simulink subsystem "Wind_Forces"  (R2026a)
settings: Solver=VariableStepAuto
undefined symbols (not defined in the file): IN, pressureLevels, uwndTable, vwndTable
settings Model: Creator=asing  LastModifiedBy=asing

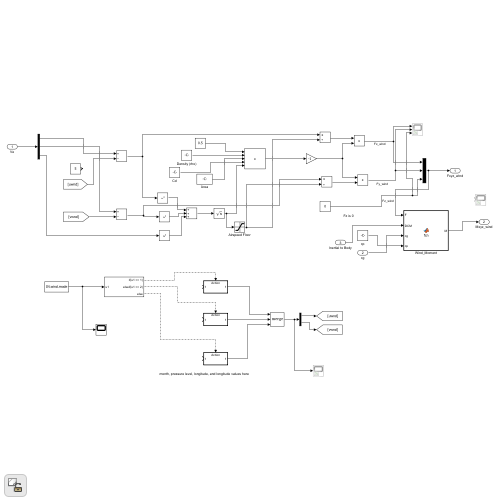
[thumbnail: Simulink's stored preview of the top-level diagram]
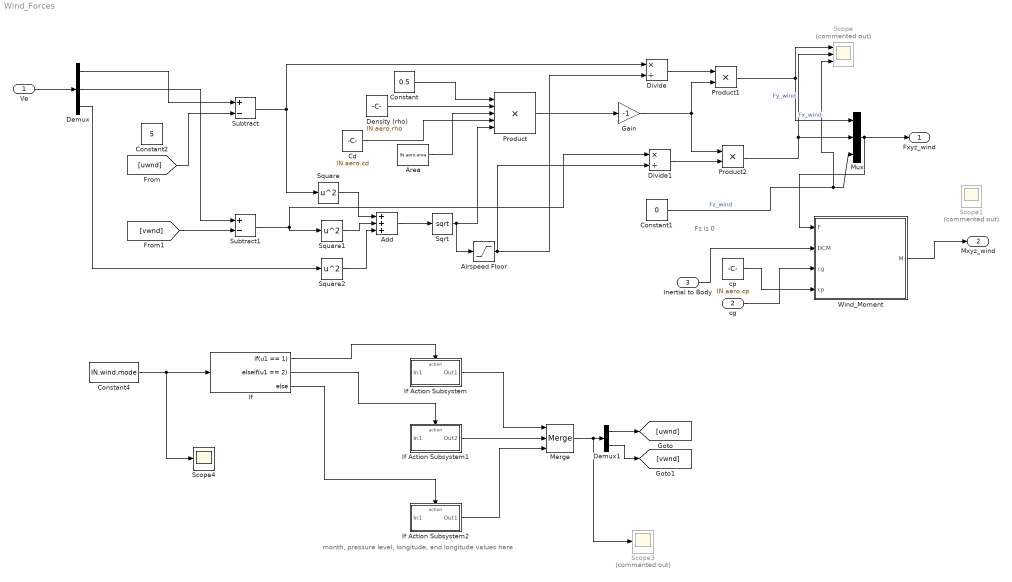
== system Wind_Forces ==
  note: month, pressure level, longitude, and longitude values here
  note: Fz is 0
  Ve : Inport
  cg : Inport  Port=2
  Inertial to Body : Inport  Port=3
  Add : Sum  Inputs=+++
  Airspeed Floor : Saturate  Description=Avoids 0/0 in the drag direction when the air-relative speed is zero (e.g. no wind at lift-off).  UpperLimit=inf  LowerLimit=1e-6
  Area : Constant  Value=IN.aero.area
  Cd : Constant  Value=IN.aero.cd
  Constant : Constant  Value=0.5
  Constant1 : Constant  Value=0
  Constant2 : Constant  Value=5
  Constant4 : Constant  Value=IN.wind.mode
  Demux : Demux  Outputs=3
  Demux1 : Demux  Outputs=2
  Density (rho) : Constant  Value=IN.aero.rho
  Divide : Product  Inputs=*/
  Divide1 : Product  Inputs=*/
  Gain : Gain  Gain=-1
  If : If  IfExpression=u1 == 1  ElseIfExpressions=u1 == 2
  If Action Subsystem : Subsystem  TreatAsAtomicUnit=on
  If Action Subsystem1 : Subsystem  TreatAsAtomicUnit=on
  If Action Subsystem2 : Subsystem  TreatAsAtomicUnit=on
  Merge : Merge  Inputs=3
  Mux : Mux  Inputs=3
  Product : Product  Inputs=5
  Product1 : Product
  Product2 : Product
  Scope : Scope  Commented=on  NumInputPorts=3
      settings: ActiveDisplayYMinimum=-3.3865408119999993  ActiveDisplayYMaximum=30.478867308  DataLoggingVariableName=ScopeData58
  Scope1 : Scope  Commented=on
      settings: ActiveDisplayYMinimum=-10.256382918668168  ActiveDisplayYMaximum=17.46231209617951  DataLoggingVariableName=ScopeData89
  Scope3 : Scope  Commented=on
      settings: ActiveDisplayYMinimum=4  ActiveDisplayYMaximum=6  DataLoggingVariableName=ScopeData90
  Scope4 : Scope
      settings: ActiveDisplayYMinimum=1  ActiveDisplayYMaximum=3  DataLoggingVariableName=ScopeData91
  Sqrt : Sqrt
  Square : Math  Operator=square
  Square1 : Math  Operator=square
  Square2 : Math  Operator=square
  Subtract : Sum  Inputs=+-
  Subtract1 : Sum  Inputs=+-
  Wind_Moment : MATLAB Function  TreatAsAtomicUnit=on
  cp : Constant  Value=IN.aero.cp
  Fxyz_wind : Outport
  Mxyz_wind : Outport  Port=2
  wires:
  If/1 -> If Action Subsystem/Action
  Mux/1 -> Fxyz_wind/1, Wind_Moment/1(F)
  [vwnd] -> Subtract1/2
  Demux/3 -> Square2/1
  Divide1/1 -> Product2/2
  Square/1 -> Add/1
  Merge/1 -> Demux1/1, Scope3/1
  Demux1/2 -> [vwnd]
  Gain/1 -> Product2/1, Product1/2
  Ve/1 -> Demux/1
  Subtract/1 -> Square/1, Divide/1
  If/2 -> If Action Subsystem1/Action
  Sqrt/1 -> Airspeed Floor/1, Product/5
  Demux1/1 -> [uwnd]
  [uwnd] -> Subtract/2
  Area/1 -> Product/3
  Square2/1 -> Add/3
  Product2/1 -> Mux/2, Scope/2  "Fy_wind"
  Constant4/1 -> If/1, Scope4/1
  Constant1/1 -> Mux/3, Scope/3  "Fz_wind"
  If/3 -> If Action Subsystem2/Action
  Product1/1 -> Mux/1, Scope/1  "Fx_wind"
  Cd/1 -> Product/4
  Subtract1/1 -> Divide1/1, Square1/1
  Density (rho)/1 -> Product/2
  If Action Subsystem/1(Out1) -> Merge/1
  If Action Subsystem2/1(Out1) -> Merge/3
  Constant/1 -> Product/1
  Demux/2 -> Subtract1/1
  If Action Subsystem1/1(Out2) -> Merge/2
  Divide/1 -> Product1/1
  Add/1 -> Sqrt/1
  Product/1 -> Gain/1
  Square1/1 -> Add/2
  Demux/1 -> Subtract/1
  Airspeed Floor/1 -> Divide1/2, Divide/2
  Inertial to Body/1 -> Wind_Moment/2(DCM)
  cg/1 -> Wind_Moment/3(cg)
  cp/1 -> Wind_Moment/4(cp)
  Wind_Moment/1(M) -> Mxyz_wind/1

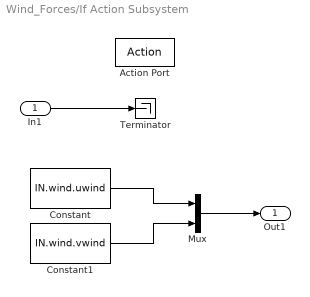
== system Wind_Forces/If Action Subsystem ==
  In1 : Inport
  Action Port : ActionPort
  Constant : Constant  Value=IN.wind.uwind
  Constant1 : Constant  Value=IN.wind.vwind
  Mux : Mux  Inputs=2
  Terminator : Terminator
  Out1 : Outport
  wires:
  Mux/1 -> Out1/1
  Constant1/1 -> Mux/2
  Constant/1 -> Mux/1
  In1/1 -> Terminator/1

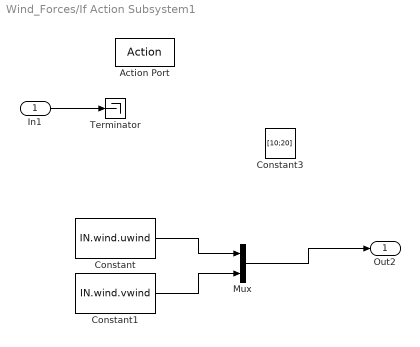
== system Wind_Forces/If Action Subsystem1 ==
  In1 : Inport
  Action Port : ActionPort
  Constant : Constant  Value=IN.wind.uwind
  Constant1 : Constant  Value=IN.wind.vwind
  Constant3 : Constant  Value=[10;20]
  Mux : Mux  Inputs=2
  Terminator : Terminator
  Out2 : Outport
  wires:
  Constant1/1 -> Mux/2
  Constant/1 -> Mux/1
  Mux/1 -> Out2/1
  In1/1 -> Terminator/1

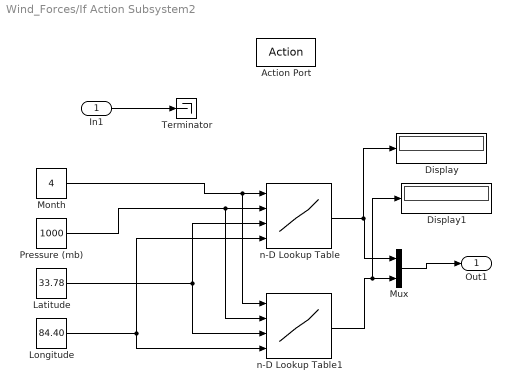
== system Wind_Forces/If Action Subsystem2 ==
  In1 : Inport
  Action Port : ActionPort
  Display : Display
  Display1 : Display
  Latitude : Constant  Value=33.78
  Longitude : Constant  Value=84.40
  Month : Constant  Value=4
  Mux : Mux  Inputs=2
  Pressure (mb) : Constant  Value=1000
  Terminator : Terminator
  n-D Lookup Table : Lookup_n-D  NumberOfTableDimensions=4  BreakpointsForDimension1=1:12  BreakpointsForDimension2=pressureLevels  BreakpointsForDimension3=[32.5 35]  BreakpointsForDimension4=[82.5 85]  Table=uwndTable  ExtrapMethod=Clip  InternalRulePriority=Speed  RndMeth=Simplest
      settings: InputPortMap=u0,u1,u2,u3
  n-D Lookup Table1 : Lookup_n-D  NumberOfTableDimensions=4  BreakpointsForDimension1=1:12  BreakpointsForDimension2=pressureLevels  BreakpointsForDimension3=[32.5 35]  BreakpointsForDimension4=[82.5 85]  Table=vwndTable  InternalRulePriority=Speed  RndMeth=Simplest
      settings: InputPortMap=u0,u1,u2,u3
  Out1 : Outport
  wires:
  Mux/1 -> Out1/1
  n-D Lookup Table1/1 -> Mux/2, Display1/1
  n-D Lookup Table/1 -> Mux/1, Display/1
  Longitude/1 -> n-D Lookup Table/4, n-D Lookup Table1/4
  In1/1 -> Terminator/1
  Latitude/1 -> n-D Lookup Table/3, n-D Lookup Table1/3
  Pressure (mb)/1 -> n-D Lookup Table/2, n-D Lookup Table1/2
  Month/1 -> n-D Lookup Table/1, n-D Lookup Table1/1

== matlab function Wind_Forces/Wind_Moment ==
  data: F input; M output; DCM input; cg input; cp input
function M = fcn(F, DCM, cg, cp)
% Wind moment about the CG in inertial axes (the model rotates it to
% body axes with the DCM, like the force): r x F, with the centre of
% pressure cp metres from the base along the body x axis
r = DCM' * [cp - cg(1); 0; 0];
M = cross(r, F(:));
end
